simulink model "MotionLoopTest"  (R2026b)
settings: Solver=ode4  StopTime=fixtureCfg.Duration  FixedStep=experimentCfg.Step
PostLoadFcn:
  | addpath(fullfile(fileparts(fileparts(fileparts(fileparts(fileparts(get_param(bdroot,'FileName')))))),'docs','scripts'));initialize_motor_paths();initialize_motor_model(bdroot);
model workspace (MAT data in the model file):
  currentCfg.Ts = 0.0001
  currentCfg.BandwidthHz = 500
  currentCfg.Kpd = 3.14159265359
  currentCfg.Kpq = 3.76991118431
  currentCfg.Kid = 1570.79632679
  currentCfg.Kiq = 1570.79632679
  currentCfg.Kaw = 1000
  deadtimeCfg.DeadTime = 2e-06
  deadtimeCfg.DeviceDrop = 0
  deadtimeCfg.CurrentBlend = 0.1
  deadtimeCfg.ModelEnable = 0
  deadtimeCfg.CompensationEnable = 0
  deadtimeCfg.CompensationScale = 1
  deadtimeCfg.SwitchingStep = 1e-07
  experimentCfg.Step = 5e-06
  experimentCfg.LogTs = 0.0001
  experimentCfg.Duration = 1.5
  experimentCfg.Mode = 2
  experimentCfg.UseInverter = 1
  experimentCfg.UseTiming = 1
  experimentCfg.UseMechanical = 1
  experimentCfg.ImposedElectricalSpeed = 0
  experimentCfg.IdReference = 0
  experimentCfg.IqReference = 2
  experimentCfg.IqInitial = 0
  experimentCfg.SpeedReference = 40
  experimentCfg.SpeedInitial = 0
  experimentCfg.PositionReference = 1
  experimentCfg.PositionInitial = 0
  experimentCfg.CommandTime = 0.05
  experimentCfg.LoadTorque = 0.1
  experimentCfg.LoadTime = 0.35
  experimentCfg.Enable = 1
  experimentCfg.Reset = 0
  feedforwardCfg.Enable = 0
  feedforwardCfg.ParameterScale = 1
  fixtureCfg.Ts = 0.0001
  fixtureCfg.Duration = 0.03
  fixtureCfg.SolverStep = 5e-06
  fixtureCfg.PositionReference = 1
  fixtureCfg.PositionFeedback = 0
  fixtureCfg.SpeedReference = 20
  fixtureCfg.CommandTime = 0.003
  fixtureCfg.SpeedFeedback = 0
  fixtureCfg.SpeedFeedforward = 0
  fixtureCfg.Inputs = [1 1 1 1 1 1 1 1 1 1 1 1 ... (1505 elements, 301x5)]
  inverterCfg.Vdc = 48
  inverterCfg.MinDuty = 0.02
  inverterCfg.PwmTs = 0.0001
  inverterCfg.LinearLimit = 26.6043004043
  motionCfg.Ts = 0.001
  motionCfg.NaturalFrequency = 20
  motionCfg.Damping = 0.9
  motionCfg.Kt = 0.21
  motionCfg.Kp = 0.0852380952381
  motionCfg.Ki = 0.952380952381
  motionCfg.Kaw = 20
  motionCfg.PositionKp = 8
  motionCfg.SpeedLimit = 80
  motionCfg.AccelerationLimit = 200
  motionCfg.CurrentLimit = 8
  pmsmCfg.Rs = 0.5
  pmsmCfg.Ld = 0.001
  pmsmCfg.Lq = 0.0012
  pmsmCfg.Flux = 0.035
  pmsmCfg.PolePairs = 4
  pmsmCfg.J = 0.0005
  pmsmCfg.B = 0.0001
  pmsmCfg.Id0 = 0
  pmsmCfg.Iq0 = 0
  pmsmCfg.Speed0 = 0
  pmsmCfg.Position0 = 0
  testStim.time = []
  testStim.signals.values = [1 1 1 1 1 1 1 1 1 1 1 1 ... (1505 elements, 301x5)]
  testStim.signals.dimensions = 5
  timingCfg.Ts = 0.0001
  timingCfg.FeedbackTicks = 1
  timingCfg.ActuationTicks = 1
libraries: MotionControl x2
settings Model: Creator=24322  LastModifiedBy=24322

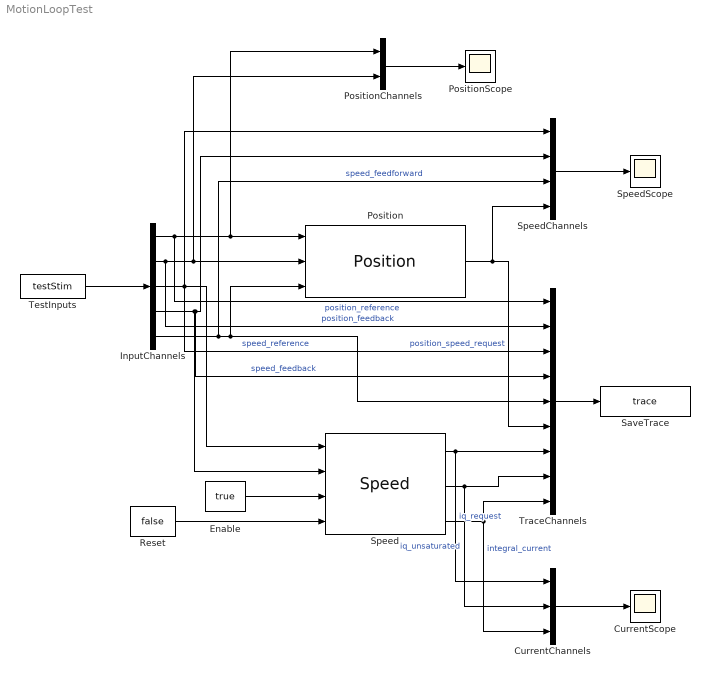
== system MotionLoopTest ==
  CurrentChannels : Mux  Inputs=3
  CurrentScope : Scope
      settings: Title=Current  YLabel=A
  Enable : Constant  Value=true  OutDataTypeStr=boolean
  InputChannels : Demux  Outputs=5
  Position : MotionControl/Position  SystemSampleTime=-1  VariantActivationTime=update diagram  EmptyChoice=off  PassThrough=off  PassThroughVariantControl=(default)  EmptyChoiceVariantControl=(default)  AllowFlexibleInterface=on  Latency=0  AutoFrameSizeCalculation=off
  PositionChannels : Mux  Inputs=2
  PositionScope : Scope
      settings: Title=Position  YLabel=rad
  Reset : Constant  Value=false  OutDataTypeStr=boolean
  SaveTrace : ToWorkspace  VariableName=trace  SaveFormat=Structure With Time  SampleTime=experimentCfg.LogTs
  Speed : MotionControl/Speed  SystemSampleTime=-1  VariantActivationTime=update diagram  EmptyChoice=off  PassThrough=off  PassThroughVariantControl=(default)  EmptyChoiceVariantControl=(default)  AllowFlexibleInterface=on  Latency=0  AutoFrameSizeCalculation=off
  SpeedChannels : Mux
  SpeedScope : Scope
      settings: Title=Speed  YLabel=rad/s
  TestInputs : FromWorkspace  VariableName=testStim  SampleTime=currentCfg.Ts  Interpolate=off  OutputAfterFinalValue=Holding final value
  TraceChannels : Mux  Inputs=9
  wires:
  CurrentChannels/1 -> CurrentScope/1
  SpeedChannels/1 -> SpeedScope/1
  PositionChannels/1 -> PositionScope/1
  Speed/3 -> TraceChannels/9, CurrentChannels/3  "integral_current"
  Speed/2 -> TraceChannels/8, CurrentChannels/2  "iq_unsaturated"
  Speed/1 -> TraceChannels/7, CurrentChannels/1  "iq_request"
  Position/1 -> TraceChannels/6, SpeedChannels/4  "position_speed_request"
  TraceChannels/1 -> SaveTrace/1
  Reset/1 -> Speed/4
  Enable/1 -> Speed/3
  InputChannels/4 -> TraceChannels/4, SpeedChannels/2, Speed/2  "speed_feedback"
  InputChannels/3 -> Speed/1, TraceChannels/3, SpeedChannels/1  "speed_reference"
  InputChannels/5 -> Position/3, TraceChannels/5, SpeedChannels/3  "speed_feedforward"
  InputChannels/2 -> Position/2, PositionChannels/2, TraceChannels/2  "position_feedback"
  InputChannels/1 -> PositionChannels/1, Position/1, TraceChannels/1  "position_reference"
  TestInputs/1 -> InputChannels/1
